simulink model "ATOM_parking_chain"  (R2026a)
settings: Solver=ode4  StopTime=100  FixedStep=0.01
StopFcn:
  | % Put every new figure in the same MATLAB Figures window as a docked tab.
  | set(groot, 'defaultFigureWindowStyle', 'docked');
  | 
  | if exist('costmap_active', 'var') && ...
  |         exist('vehicle', 'var') && ...
  |         exist('parking_path', 'var') && ...
  |         ~isempty(parking_path)
  | 
  |     plotPlan(costmap_active, vehicle, parking_path);
  | 
  | else
  | 
  |     warning('No valid parking path is available for plotting.');
  | 
  | end
  | 
  | PlotControllerReferences( ...
  |     out.controller_reference_log);
  | 
  | PlotControllerTracking( ...
  |     out.controller_tracking_log);
undefined symbols (not defined in the file): lateral, longitudinal, stanley, vehicle
(part 8 of 11)

== matlab function ATOM_parking_chain/Vehicle_Model2/Vehicle Dynamics/MATLAB Function ==
  data: state input Bus: VehicleInternalStateBus size=1; d_state output Bus: VehicleInternalStateBus size=1; command input Bus: ControlCMDBus size=1; veh input; rear_steering_command input
function d_state = vehicleDynamics(state, command, veh, rear_steering_command)

%%%%%%%%%%%%%%%%%%%%%%%%%%%%%%%%%%%%%%
%%%%%%%%%%%%%%%%%%%%%%%%%%%%%%%%%%%%%%
% Description:
% This vehicleDynamics model follows DELAY_STEER_ACC_GEARED
% model, it doesn't presents a model for gear management
% since its not something we're going to modify on Autoware for 4WS
% implementation.
%
% Inputs:
% - state: VehicleInternalStateBus. It contains the state of the vehicle
%          at time instant t. 
% - command: /control/command/control_cmd topic --> ControlCMDBus.
%          It contains the desired acc and steering commands coming from
%          the control region.
%
% - Parameters
% - vehicle: vehicle parameters struct defined in vehicleParameters.m.

% Outputs: 
% - d_state: It contains the derivative of the state of the vehicle at time
%          instant t+1.
%%%%%%%%%%%%%%%%%%%%%%%%%%%%%%%%%%%%%%
%%%%%%%%%%%%%%%%%%%%%%%%%%%%%%%%%%%%%%


% inside MATLAB Function: input is veh_in (1xN double)
v = veh; % 1xN numeric row

vehicle.param.wheel_radius    = v(1);
vehicle.param.wheel_width     = v(2);
vehicle.param.wheel_base      = v(3);
vehicle.param.wheel_tread     = v(4);
vehicle.param.front_overhang  = v(5);
vehicle.param.rear_overhang   = v(6);
vehicle.param.left_overhang   = v(7);
vehicle.param.right_overhang  = v(8);
vehicle.param.vehicle_height  = v(9);
vehicle.param.max_steer_angle = v(10);

% decode integer-coded enums (example)
vehicle.sim.vehicle_model_type = int32(v(11));    % or map to strings if needed
vehicle.sim.initialize_source  = int32(v(12));

vehicle.sim.timer_sampling_time_ms = v(13);
vehicle.sim.add_measurement_noise = logical(v(14));
vehicle.sim.vel_lim        = v(15);
vehicle.sim.vel_rate_lim   = v(16);
vehicle.sim.steer_lim      = v(17);
vehicle.sim.steer_rate_lim = v(18);
vehicle.sim.acc_time_delay = v(19);
vehicle.sim.acc_time_constant = v(20);
vehicle.sim.steer_time_delay   = v(21);
vehicle.sim.steer_time_constant= v(22);
vehicle.sim.x_stddev = v(23);
vehicle.sim.y_stddev = v(24);
vehicle.sim.steer_dead_band = v(25);
vehicle.sim.steer_bias = v(26);
vehicle.sim.debug_acc_scaling_factor = v(27);
vehicle.sim.debug_steer_scaling_factor = v(28);

% Parameter for 4WS
vehicle.param.rear_steering_ratio = veh(29);
rear_steering_ratio = vehicle.param.rear_steering_ratio;

%% ==========================
% Saturation function
% ===========================

sat = @(val, upper, lower) min(max(val,lower),upper);



%% ==========================
% Current state
% ===========================

vx = sat( ...
    state.vx,...
    vehicle.sim.vel_lim,...
   -vehicle.sim.vel_lim);


acc = sat( ...
    state.acc,...
    vehicle.sim.vel_rate_lim,...
   -vehicle.sim.vel_rate_lim);


yaw = state.yaw;

steer_front = state.steer_front;
steer_rear = state.steer_rear;          % Modified for 4WS  


%% ==========================
% Input commands
% ===========================

acc_des = sat( ...
    command.longitudinal.acceleration,...
    vehicle.sim.vel_rate_lim,...
   -vehicle.sim.vel_rate_lim);


acc_des = acc_des * ...
    vehicle.sim.debug_acc_scaling_factor;



steer_front_des = sat( ...
    command.lateral.steering_tire_angle,...
    vehicle.sim.steer_lim,...
   -vehicle.sim.steer_lim);


steer_front_des = steer_front_des * ...
    vehicle.sim.debug_steer_scaling_factor;

steer_rear_des = sat( ...                                            % Modified for 4WS
    rear_steering_command,...
    vehicle.sim.steer_lim,...
    -vehicle.sim.steer_lim);


steer_rear_des = steer_rear_des * ...                                % Modified for 4WS
    vehicle.sim.debug_steer_scaling_factor;



%% ==========================
% Steering dynamics
% ===========================

% getSteer() in simple_planning_simulator corresponds to state.steer
% From the phisical vehicle front_steer and rear_steer are measured.

steer_diff_front = steer_front - steer_front_des;

steer_diff_rear = steer_rear  - steer_rear_des;             % Modified for 4WS


% dead band

if steer_diff_front > vehicle.sim.steer_dead_band

    steer_diff_with_dead_band_front = ...
        steer_diff_front - vehicle.sim.steer_dead_band;


elseif steer_diff_front < -vehicle.sim.steer_dead_band

    steer_diff_with_dead_band_front = ...
        steer_diff_front + vehicle.sim.steer_dead_band;


else

    steer_diff_with_dead_band_front = 0;

end



if steer_diff_rear > vehicle.sim.steer_dead_band            % Modified for 4WS

    steer_diff_with_dead_band_rear = ...
        steer_diff_rear - vehicle.sim.steer_dead_band;


elseif steer_diff_rear < -vehicle.sim.steer_dead_band

    steer_diff_with_dead_band_rear = ...
        steer_diff_rear + vehicle.sim.steer_dead_band;


else

    steer_diff_with_dead_band_rear = 0;

end



steer_rate_front = sat( ...
    -steer_diff_with_dead_band_front / vehicle.sim.steer_time_constant,...
     vehicle.sim.steer_rate_lim,...
    -vehicle.sim.steer_rate_lim);

steer_rate_rear = sat( ...                                                  % Modified for 4WS
    -steer_diff_with_dead_band_rear / vehicle.sim.steer_time_constant,...
    vehicle.sim.steer_rate_lim,...
    -vehicle.sim.steer_rate_lim);



%% ==========================
% State derivative
% ===========================

%--------------------------------------------------------------
% 4WS kinematic bicycle model
%
% Assumptions:
%   - Pure rolling
%   - alpha_f = alpha_r = 0
%   - No tire dynamics
%   - No lateral slip dynamics
%
% beta is the geometric vehicle sideslip angle. Since Autoware defines
% reference frame of the vehicle equal to centre of the rear axle, then
% beta = steer_rear
%--------------------------------------------------------------

L = vehicle.param.wheel_base;


beta = steer_rear;                              % Modified for 4WS


vel = vx/cos(beta);                             % Modified for 4WS


yaw_rate = ...                                  % Modified for 4WS
    (vx/L) * ...
    (tan(steer_front)-tan(steer_rear));


d_state.x = vel*cos(yaw + beta);                % Modified for 4WS

d_state.y = vel*sin(yaw + beta);                % Modified for 4WS


d_state.yaw = yaw_rate;                         % Modified for 4WS


d_state.vx = acc + yaw_rate*vel*sin(beta);


d_state.steer_front = steer_rate_front;

d_state.steer_rear = steer_rate_rear;           % Modified for 4WS

d_state.acc = ...
    -(acc-acc_des)/vehicle.sim.acc_time_constant;

end

== matlab function ATOM_parking_chain/Vehicle_Model2/localization//acceleration function ==
  data: state input Bus: VehicleInternalStateBus; accel output Bus: AccelerationBus; veh input
function accel = IntStateToAccelerationState(state,veh)

L = veh(3);

vx = state.vx;
ax = state.acc;

delta_f = state.steer_front;
delta_r = state.steer_rear;

yaw_rate = (vx/L)*(tan(delta_f)-tan(delta_r));

ay = vx*yaw_rate;

accel.acceleration.linear.x = ax;
accel.acceleration.linear.y = ay;
accel.acceleration.linear.z = 0;

accel.acceleration.angular.x = 0;
accel.acceleration.angular.y = 0;
accel.acceleration.angular.z = 0;

end

== matlab function ATOM_parking_chain/time_parameterization/Time parameterization ==
  data: trajectory_in input Bus: TrajectoryDataBus size=1; reference_out output Bus: ParkingReferenceBus size=1; steer_rate_limit input
function reference_out = timeParameterization( ...
    trajectory_in,steer_rate_limit)
%#codegen
%
% Convert the 100-point spatial parking trajectory into a nominal
% time-parameterized reference trajectory.

N = 100;

%% Extract the smoothed trajectory

x_ref = trajectory_in.pose.position.x;
y_ref = trajectory_in.pose.position.y;

qz = trajectory_in.pose.orientation.qz;
qw = trajectory_in.pose.orientation.qw;

v_ref = trajectory_in.longitudinal_velocity_mps;
a_ref = trajectory_in.acceleration_mps2;

df_plan = trajectory_in.front_wheel_angle_rad;
dr_plan = trajectory_in.rear_wheel_angle_rad;

rear_angle = trajectory_in.rear_wheel_angle_rad;

%% Convert quaternion to continuous body-heading reference

psi_ref = zeros(N,1);

psi_ref(1) = 2.0*atan2(qz(1),qw(1));

for k = 2:N

    raw_heading = 2.0*atan2(qz(k),qw(k));

    heading_change = raw_heading-psi_ref(k-1);

    psi_ref(k) = ...
        raw_heading-2.0*pi*round(heading_change/(2.0*pi));
end

%% Calculate distance and nominal time

s_ref = zeros(N,1);
t_ref = zeros(N,1);

for k = 1:N-1

    dx = x_ref(k+1)-x_ref(k);
    dy = y_ref(k+1)-y_ref(k);

    ds = hypot(dx,dy);

    s_ref(k+1) = s_ref(k)+ds;

    % Convert signed body-longitudinal velocity to positive rear-axle
    % path speed.
    path_speed_current = ...
        abs(v_ref(k))/max(cos(rear_angle(k)),0.1);

    path_speed_next = ...
        abs(v_ref(k+1))/max(cos(rear_angle(k+1)),0.1);

    speed_sum = path_speed_current+path_speed_next;

    if ds <= 1e-9

        dt = 0.0;

    elseif speed_sum > 1e-6

        % ds = 0.5*(v_current+v_next)*dt
        dt = 2.0*ds/speed_sum;

    else

        % Protect against an interval whose two endpoint speeds are zero.
        fallback_path_speed = 0.05;

        dt = ds/fallback_path_speed;
    end

    t_ref(k+1) = t_ref(k)+dt;
end
N = numel(t_ref);

df_nom = zeros(size(df_plan));
dr_nom = zeros(size(dr_plan));

% Start from the planner's first steering configuration.
df_nom(1) = df_plan(1);
dr_nom(1) = dr_plan(1);

for i = 2:N

    dt = max(t_ref(i)-t_ref(i-1),0.0);
    maximum_change = steer_rate_limit*dt;

    front_difference = df_plan(i)-df_nom(i-1);
    rear_difference  = dr_plan(i)-dr_nom(i-1);

    front_change = max( ...
        -maximum_change, ...
        min(maximum_change,front_difference));

    rear_change = max( ...
        -maximum_change, ...
        min(maximum_change,rear_difference));

    df_nom(i) = df_nom(i-1)+front_change;
    dr_nom(i) = dr_nom(i-1)+rear_change;

end

reference_out.t_ref   = t_ref;
reference_out.s_ref   = s_ref;
reference_out.x_ref   = x_ref;
reference_out.y_ref   = y_ref;
reference_out.psi_ref = psi_ref;
reference_out.v_ref   = v_ref;
reference_out.a_ref   = a_ref;
% Temporary pass-through. The next step will make these rate-feasible.
reference_out.df_nom = df_nom;
reference_out.dr_nom = dr_nom;
end

== matlab function ATOM_parking_chain/Parking Scenario/Costmap generation: empty occupancy grid/MATLAB Function ==
  data: veh input; costmap output Bus: OccupancyGridBus; start_pose output; goal_pose output
function [costmap, start_pose, goal_pose] = costmapEmptyLot(veh) %#ok<INUSD>
%COSTMAPEMPTYLOT  Empty lot - no objects layer. The reference case:
% whatever the planner does here is forced by the turning radius alone,
% not by obstacles.
%
% veh is unused (no parked cars to size) but kept so all costmap blocks
% have identical ports and can be rewired freely.

persistent occ

res = 0.3;   W = 234;   H = 234;
origin_x = -(W/2)*res;
origin_y = -(H/2)*res;

if isempty(occ)
    [IX, IY] = meshgrid(0:W-1, 0:H-1);
    X = origin_x + IX*res;
    Y = origin_y + IY*res;

    lot_x = [-15  15  15 -15];
    lot_y = [-12 -12  12  12];
    occ = ones(H,W);
    occ(inpolygon(X, Y, lot_x, lot_y)) = 0;
end

start_pose = [-8, 0, 0];
goal_pose  = [ 0, 5, pi/2];

costmap.info.resolution           = res;
costmap.info.width                = uint32(W);
costmap.info.height               = uint32(H);
costmap.info.origin.position.x    = origin_x;
costmap.info.origin.position.y    = origin_y;
costmap.info.origin.position.z    = 0;
costmap.info.origin.orientation.x = 0;
costmap.info.origin.orientation.y = 0;
costmap.info.origin.orientation.z = 0;
costmap.info.origin.orientation.w = 1;
costmap.data                      = int8(occ*100);
end

== matlab function ATOM_parking_chain/Vehicle_Model2/localization//kinematic_state function ==
  data: state input Bus: VehicleInternalStateBus; kinematic output Bus: KinematicStateBus; veh input
function kinematic = IntStateToKinematicState(state, veh)


%% Vehicle parameters

L = veh(3);


%% Current state

x = state.x;
y = state.y;
yaw = state.yaw;



% NOTE:
% vx is the longitudinal velocity expressed in the vehicle body frame
% (base_link located at the center of the rear axle).
% The vehicle speed magnitude is reconstructed as
%
%   v = vx / cos(delta_r)
%
% under the pure-rolling assumption (alpha_f = alpha_r = 0).

vx = state.vx;

steer_front = state.steer_front;
steer_rear  = state.steer_rear;


%% Pose

kinematic.pose.position.x = x;
kinematic.pose.position.y = y;
kinematic.pose.position.z = 0;


[qx,qy,qz,qw] = yawToQuaternion(yaw);

% quaternion from yaw only

kinematic.pose.orientation.x = qx;
kinematic.pose.orientation.y = qy;
kinematic.pose.orientation.z = qz;
kinematic.pose.orientation.w = qw;



%% Twist

% Body frame velocity

kinematic.twist.linear.x = vx;

kinematic.twist.linear.y = ...              % Modified for 4WS considering beta = steer_rear
    vx*tan(steer_rear);

kinematic.twist.linear.z = 0;



% Angular velocity

kinematic.twist.angular.x = 0;
kinematic.twist.angular.y = 0;

kinematic.twist.angular.z = ...
    (vx/L) * ...
    (tan(steer_front)-tan(steer_rear));


end

== matlab function ATOM_parking_chain/Parking Scenario/Costmap generation: corridor occupancy grid/MATLAB Function ==
  data: veh input; costmap output Bus: OccupancyGridBus; start_pose output; goal_pose output
function [costmap, start_pose, goal_pose] = costmapNarrowCorridor(veh) %#ok<INUSD>
%COSTMAPNARROWCORRIDOR  8 m wide corridor.
%
% The planner turns in 5.47 m and the car is 2.66 m wide with its margin,
% so this corridor allows driving through but not turning around.
% Default task is a straight transit, which succeeds.
%
% To make it the limit case, change goal_pose heading to -pi/2 - a U-turn.
% That is expected to FAIL with a 5.47 m radius, and it is exactly the
% case a tighter turning circle would change.

persistent occ

res = 0.3;   W = 234;   H = 234;
origin_x = -(W/2)*res;
origin_y = -(H/2)*res;

if isempty(occ)
    [IX, IY] = meshgrid(0:W-1, 0:H-1);
    X = origin_x + IX*res;
    Y = origin_y + IY*res;

    lot_x = [ -4   4   4  -4];
    lot_y = [-12 -12  12  12];
    occ = ones(H,W);
    occ(inpolygon(X, Y, lot_x, lot_y)) = 0;
end

start_pose = [0, -8, pi/2];
goal_pose  = [0,  6, pi/2];

costmap.info.resolution           = res;
costmap.info.width                = uint32(W);
costmap.info.height               = uint32(H);
costmap.info.origin.position.x    = origin_x;
costmap.info.origin.position.y    = origin_y;
costmap.info.origin.position.z    = 0;
costmap.info.origin.orientation.x = 0;
costmap.info.origin.orientation.y = 0;
costmap.info.origin.orientation.z = 0;
costmap.info.origin.orientation.w = 1;
costmap.data                      = int8(occ*100);
end

== matlab function ATOM_parking_chain/Parking Scenario/Costmap generation: parking scenario beside a lane/MATLAB Function ==
  settings: updateMethod=DISCRETE
  data: veh input; costmap output Bus: OccupancyGridBus; start_pose output; goal_pose output
function [costmap, start_pose, goal_pose] = costmapDoubleRowLot(veh)
%COSTMAPDOUBLEROWLOT  Two rows of bays with a realistic aisle between them.
%
% Harder than the single-row lot: the car must enter the bay from an 8.6 m
% aisle with a 5.47 m turning radius, so it cannot swing in with one arc.
%
% Reproduces autoware_costmap_generator geometry:
%   grid_resolution 0.3, grid_length_x/y 70.0, expand_polygon_size 0.5

persistent occ

res = 0.3;   W = 234;   H = 234;
origin_x = -(W/2)*res;
origin_y = -(H/2)*res;

bay_x   = (-2:2)*3.6;          % 5 bays per row, 3.6 m pitch
row_y   = 6.0;                 % rows at y = +6 and y = -6  -> 8.6 m aisle
free_bay = 3;                  % the empty one, top row (x = 0)

if isempty(occ)
    [IX, IY] = meshgrid(0:W-1, 0:H-1);
    X = origin_x + IX*res;
    Y = origin_y + IY*res;

    % the lot, carved out of the wall
    lot_x = [-12  12  12 -12];
    lot_y = [ -9  -9   9   9];
    occ = ones(H,W);
    occ(inpolygon(X, Y, lot_x, lot_y)) = 0;

    car_len = veh(5) + veh(3) + veh(6);
    car_wid = veh(4) + veh(7) + veh(8);
    expand  = 0.5;
    L = car_len + expand;
    D = car_wid + expand;

    for k = 1:5
        % top row, one bay left empty
        if k ~= free_bay
            qx = [ D/2 -D/2 -D/2  D/2] + bay_x(k);
            qy = [ L/2  L/2 -L/2 -L/2] + row_y;
            occ(inpolygon(X, Y, qx, qy)) = 1;
        end
        % bottom row, fully occupied
        qx = [ D/2 -D/2 -D/2  D/2] + bay_x(k);
        qy = [ L/2  L/2 -L/2 -L/2] - row_y;
        occ(inpolygon(X, Y, qx, qy)) = 1;
    end
end

% --- the poses that belong to this scene ---------------------------------
start_pose = [-8, 0, 0];                    % in the aisle, heading east
goal_pose  = [ 0, row_y , pi/2 + pi];       % nose-in, top row, x = 0

costmap.info.resolution           = res;
costmap.info.width                = uint32(W);
costmap.info.height               = uint32(H);
costmap.info.origin.position.x    = origin_x;
costmap.info.origin.position.y    = origin_y;
costmap.info.origin.position.z    = 0;
costmap.info.origin.orientation.x = 0;
costmap.info.origin.orientation.y = 0;
costmap.info.origin.orientation.z = 0;
costmap.info.origin.orientation.w = 1;
costmap.data                      = int8(occ*100);
end

== matlab function ATOM_parking_chain/Parking Scenario/Costmap generation: complex parking situation/MATLAB Function ==
  settings: updateMethod=DISCRETE
  data: veh input; costmap output Bus: OccupancyGridBus; start_pose output; goal_pose output
function [costmap, start_pose, goal_pose] = ...
    costmapRoadsideParallelParking(veh)
%COSTMAPROADSIDEPARALLELPARKING
% A straight road with one parallel parking slot on its upper side.
%
% veh is the numeric vehicle-parameter vector:
% veh(3) = wheelbase
% veh(4) = wheel tread
% veh(5) = front overhang
% veh(6) = rear overhang
% veh(7) = left overhang
% veh(8) = right overhang

persistent occ

%% Grid

res = 0.3;
W = 234;
H = 234;

origin_x = -(W/2)*res;
origin_y = -(H/2)*res;

%% Vehicle dimensions

wheelbase      = veh(3);
wheel_tread    = veh(4);
front_overhang = veh(5);
rear_overhang  = veh(6);
left_overhang  = veh(7);
right_overhang = veh(8);

car_len = front_overhang + wheelbase + rear_overhang;
car_wid = wheel_tread + left_overhang + right_overhang;

%% Parking-scene parameters

% Obstacle inflation, matching the costmap generator
expand = 0.5;

parked_car_len = car_len + expand;
parked_car_wid = car_wid + expand;

% Road boundaries
road_x_min = -14;
road_x_max =  14;
road_y_min = -2.2;
road_y_max =  2.2;

% Tight empty-slot length
% With the current ATOM dimensions, this gives about 0.4 m clearance
% at each end for the inflated ego footprint.
slot_extra_length = 2.0;%1.3
slot_length = car_len + slot_extra_length;
slot_center_x = 0;

% Parking strip beside the road
parking_strip_width = parked_car_wid + 0.6;
parking_y = road_y_max + parking_strip_width/2;
parking_y_max = road_y_max + parking_strip_width;

% Small separation between parked vehicles outside the empty slot
inter_car_gap = 0.3;

%% Generate the occupancy grid

if isempty(occ)

    [IX,IY] = meshgrid(0:W-1,0:H-1);

    X = origin_x + IX*res;
    Y = origin_y + IY*res;

    % Begin with the whole map occupied
    occ = ones(H,W);

    % Create the road and its parking strip
    free_x = [ ...
        road_x_min, road_x_max, ...
        road_x_max, road_x_min];

    free_y = [ ...
        road_y_min, road_y_min, ...
        parking_y_max, parking_y_max];

    occ(inpolygon(X,Y,free_x,free_y)) = 0;

    %% Parked-car positions

    % Distance from the slot centre to either adjacent car centre
    adjacent_offset = ...
        (slot_length + parked_car_len)/2;

    % Two cars on each side of the empty slot
    parked_car_x = [ ...
        -adjacent_offset - parked_car_len - inter_car_gap, ...
        -adjacent_offset, ...
         adjacent_offset, ...
         adjacent_offset + parked_car_len + inter_car_gap];

    %% Add the parked cars

    for k = 1:length(parked_car_x)

        car_x = parked_car_x(k);

        % The cars are parallel to the road:
        % length along x and width along y
        qx = [ ...
            -parked_car_len/2, ...
             parked_car_len/2, ...
             parked_car_len/2, ...
            -parked_car_len/2] + car_x;

        qy = [ ...
            -parked_car_wid/2, ...
            -parked_car_wid/2, ...
             parked_car_wid/2, ...
             parked_car_wid/2] + parking_y;

        occ(inpolygon(X,Y,qx,qy)) = 1;
    end
end

%% Starting pose

% Rear-axle centre, travelling east along the road
start_pose = [-10, 0, 0];%;%%;

%% Goal pose

% The parking slot is defined using its geometric centre, but Autoware's
% vehicle pose is the rear-axle centre.
body_center_from_rear_axle = ...
    (wheelbase + front_overhang - rear_overhang)/2;

goal_pose = [ ...
    slot_center_x - body_center_from_rear_axle, ...
    parking_y, ...
    0];

%% Costmap message

costmap.info.resolution = res;
costmap.info.width      = uint32(W);
costmap.info.height     = uint32(H);

costmap.info.origin.position.x = origin_x;
costmap.info.origin.position.y = origin_y;
costmap.info.origin.position.z = 0;

costmap.info.origin.orientation.x = 0;
costmap.info.origin.orientation.y = 0;
costmap.info.origin.orientation.z = 0;
costmap.info.origin.orientation.w = 1;

costmap.data = int8(occ*100);

end

== matlab function ATOM_parking_chain/Parking Scenario/Costmap generation: obstacle/MATLAB Function ==
  settings: updateMethod=DISCRETE
  data: veh input; costmap output Bus: OccupancyGridBus; start_pose output; goal_pose output
function [costmap, start_pose, goal_pose] = costmapSingleObstacle(veh) %#ok<INUSD>
%COSTMAPSINGLEOBSTACLE  Open area with one obstacle blocking the direct route.
% Paste this function into the connected costmap MATLAB Function block.
% Poses refer to the rear-axle centre; headings are in radians.
% Keep the vehicle input so the existing Simulink connections still match.

% Fixed dimensions match the existing OccupancyGrid bus.
res = 0.2;
W = 234;
H = 234;
origin_x = -(W/2)*res;
origin_y = -(H/2)*res;

% Editable scene dimensions [m].
area_x_min = -14;
area_x_max =  14;
area_y_min =  -8;
area_y_max =   8;

obstacle_center_x = 0;
obstacle_center_y = 0;
obstacle_length = 3;  % Along x.
obstacle_width  = 5;  % Along y.

start_pose = [-8, 0, 0];
goal_pose  = [ 8, 0, 0];

% Rebuild each call so changes cannot leave an old persistent map active.
[IX, IY] = meshgrid(0:W-1, 0:H-1);
X = origin_x + IX*res;
Y = origin_y + IY*res;

% Outside the open area is occupied; inside is free.
occupied = ~(X >= area_x_min & X <= area_x_max & ...
             Y >= area_y_min & Y <= area_y_max);

% The physical obstacle is added without extra inflation. collisionCheck
% already includes the planner's vehicle-shape margin.
obstacle = abs(X-obstacle_center_x) <= obstacle_length/2 & ...
           abs(Y-obstacle_center_y) <= obstacle_width/2;
occupied = occupied | obstacle;

costmap.info.resolution = res;
costmap.info.width  = uint32(W);
costmap.info.height = uint32(H);

costmap.info.origin.position.x = origin_x;
costmap.info.origin.position.y = origin_y;
costmap.info.origin.position.z = 0;
costmap.info.origin.orientation.x = 0;
costmap.info.origin.orientation.y = 0;
costmap.info.origin.orientation.z = 0;
costmap.info.origin.orientation.w = 1;

% Preserve the existing H-by-W int8 bus payload: free=0, occupied=100.
costmap.data = int8(occupied) .* int8(100);
end
